simulink model "lab4_pid_kalman"  (R2025b)
settings: Solver=ode45  StartTime=0.0  StopTime=25  MaxStep=0.02  RelTol=1e-3
undefined symbols (not defined in the file): Akal, Bkal, C0, Kpid, num1, Rpid, T, T1, T2
settings Model: Creator=Nickolay  LastModifiedBy=Nickolay

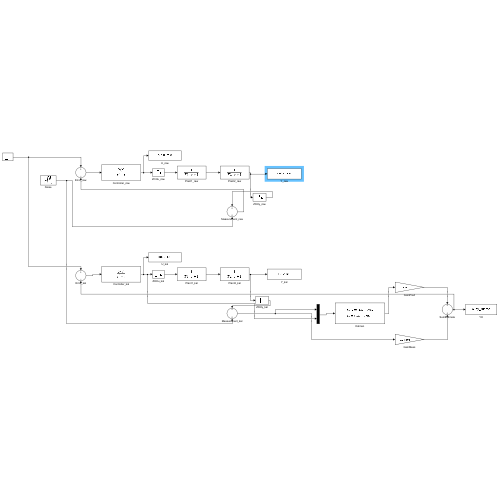
[thumbnail: Simulink's stored preview of the top-level diagram]
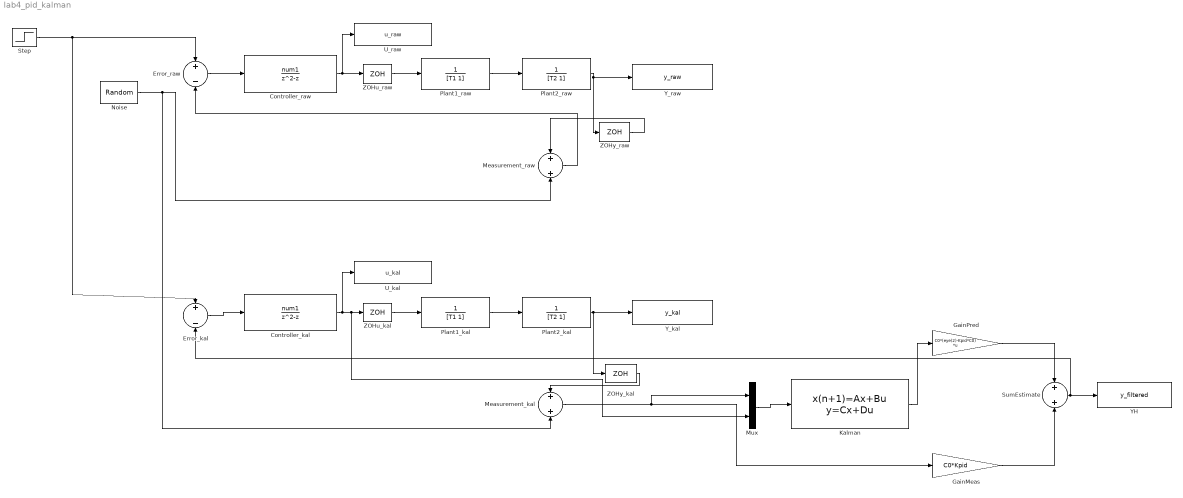
== system lab4_pid_kalman ==
  Controller_kal : DiscreteTransferFcn  Numerator=num1  Denominator=[1 -1 0]  SampleTime=T
  Controller_raw : DiscreteTransferFcn  Numerator=num1  Denominator=[1 -1 0]  SampleTime=T
  Error_kal : Sum  Inputs=+-
  Error_raw : Sum  Inputs=+-
  GainMeas : Gain  Gain=C0*Kpid
  GainPred : Gain  Gain=C0*(eye(2)-Kpid*C0)  Multiplication=Matrix(K*u)
  Kalman : DiscreteStateSpace  A=Akal  B=Bkal  C=eye(2)  D=zeros(2,2)  InitialCondition=[0;0]  SampleTime=T
  Measurement_kal : Sum
  Measurement_raw : Sum
  Mux : Mux  Inputs=2
  Noise : RandomNumber  Variance=Rpid  Seed=77  SampleTime=T
  Plant1_kal : TransferFcn  Denominator=[T1 1]
  Plant1_raw : TransferFcn  Denominator=[T1 1]
  Plant2_kal : TransferFcn  Denominator=[T2 1]
  Plant2_raw : TransferFcn  Denominator=[T2 1]
  Step : Step  Time=0  SampleTime=0
  SumEstimate : Sum
  U_kal : ToWorkspace  VariableName=u_kal  SaveFormat=Timeseries  SampleTime=-1
  U_raw : ToWorkspace  VariableName=u_raw  SaveFormat=Timeseries  SampleTime=-1
  YH : ToWorkspace  VariableName=y_filtered  SaveFormat=Timeseries  SampleTime=-1
  Y_kal : ToWorkspace  VariableName=y_kal  SaveFormat=Timeseries  SampleTime=-1
  Y_raw : ToWorkspace  VariableName=y_raw  SaveFormat=Timeseries  SampleTime=-1
  ZOHu_kal : ZeroOrderHold  SampleTime=T
  ZOHu_raw : ZeroOrderHold  SampleTime=T
  ZOHy_kal : ZeroOrderHold  SampleTime=T
  ZOHy_raw : ZeroOrderHold  SampleTime=T
  wires:
  Step/1 -> Error_raw/1, Error_kal/1
  Error_raw/1 -> Controller_raw/1
  Controller_raw/1 -> U_raw/1, ZOHu_raw/1
  ZOHu_raw/1 -> Plant1_raw/1
  Plant1_raw/1 -> Plant2_raw/1
  Plant2_raw/1 -> Y_raw/1, ZOHy_raw/1
  ZOHy_raw/1 -> Measurement_raw/1
  Noise/1 -> Measurement_raw/2, Measurement_kal/2
  Measurement_raw/1 -> Error_raw/2
  Error_kal/1 -> Controller_kal/1
  Controller_kal/1 -> ZOHu_kal/1, Mux/2, U_kal/1
  ZOHu_kal/1 -> Plant1_kal/1
  Plant1_kal/1 -> Plant2_kal/1
  Plant2_kal/1 -> Y_kal/1, ZOHy_kal/1
  ZOHy_kal/1 -> Measurement_kal/1
  Measurement_kal/1 -> Mux/1, GainMeas/1
  Mux/1 -> Kalman/1
  Kalman/1 -> GainPred/1
  GainPred/1 -> SumEstimate/1
  GainMeas/1 -> SumEstimate/2
  SumEstimate/1 -> Error_kal/2, YH/1
